simulink model "absbrake"  (R2024a)
settings: Solver=FixedStepAuto  StartTime=0.0  StopTime=20  FixedStep=0.01  MaxStep=.01  RelTol=1e-3  AbsTol=1e-6
PreLoadFcn:
  | % Load initialization data
  | 
  | sldemo_absdata;
values from neighbouring files (symbols this model uses):
  g = 9.8    [final_abs_code.m]
  J = 5    [final_abs_code.m]
  Kf = 1    [final_abs_code.m]
  m = 400    [final_abs_code.m]
  mu_dry = [0.1 0.3 0.6 0.85 0.9 0.9 0.85 0.7 0.3 0.15 0.1]    [final_abs_code.m]
  mu_icy = [0 0.08 0.10 0.095 0.09 0.088 0.085 0.083 0.08 0.079 0.078 0.077 0.076 0.0755 0.075 0.0745 0.074 0.0735 0.073 0.0725 0.072]    [final_abs_code.m]
  mu_wet = [0 0.68 0.70 0.68 0.65 0.63 0.62 0.61 0.60 0.59 0.58 0.57 0.565 0.56 0.555 0.55 0.548 0.546 0.544 0.542 0.54]    [final_abs_code.m]
  Rr = 0.3    [final_abs_code.m]
  slip_dry = [0 0.05 0.1 0.13 0.15 0.17 0.2 0.3 0.5 0.7 1.0]    [final_abs_code.m]
  slip_icy = [0 0.05 0.10 0.15 0.20 0.25 0.30 0.35 0.40 0.45 0.50 0.55 0.60 0.65 0.70 0.75 0.80 0.85 0.90 0.95 1.0]    [final_abs_code.m]
  slip_wet = [0 0.05 0.10 0.15 0.20 0.25 0.30 0.35 0.40 0.45 0.50 0.55 0.60 0.65 0.70 0.75 0.80 0.85 0.90 0.95 1.0]    [final_abs_code.m]
  v0 = 40    [final_abs_code.m]
undefined symbols (not defined in the file or in its folder): DiscIntNeverNeededParam
libraries: fuzblock x1, slpidlib x1
CloseFcn:
  | % Close the plots that are still open
  | h = findobj(0, 'Name', 'ABS Speeds');
  | if ~isempty(h),
  |   close(h);
  | end;
  | 
  | h = findobj(0, 'Name', 'ABS Slip');
  | if ~isempty(h),
  |   close(h);
  | end;
  | 
  | % Clear initial conditions data to avoid cluttering the workspace
  | 
  | clear g v0 Rr Kf m PBmax TB I slip mu ctrl h;
Description:
  | Modeling an Anti-Lock Braking System (ABS)
  | 
  | *Summary*
  | 
  | This example describes a simple model for an Anti-Lock Braking System
  | (ABS). The model simulates the dynamic behavior of a vehicle
  | under hard braking conditions. The model represents a single wheel, which
  | may be replicated a number of times to create a model for a multi-wheel
  | vehicle.
  | 
  | This model uses the signal logging feature in Simulink(R). You log signals to the
  | MATLAB(R) workspace where you can analyze and view them. You can view
  | the code in sldemo_absbrakeplots.m to see how this is done.
  | 
  | In this model, the wheel speed is calculated in a separate component
  | named sldemo_wheelspeed_absbrake.
  | This component is then referenced using a Model block.  Note that both the
  | top model and the referenced model use a variable step solver, so Simulink
  | will track zero-crossings in the referenced model.
settings Model: FPTRunName=Active  ModifiedByFormat=The MathWorks, Inc.  Creator=The MathWorks, Inc.  LastModifiedBy=The MathWorks, Inc.
settings SolverCC: AutoScaleAbsTol=off  AlgebraicLoopSolver=TrustRegion  MaxZcPerStep=1
settings DataIOCC: SaveFormat=Array  SaveOutput=off  SaveTime=off  ReturnWorkspaceOutputs=off  TimeSaveName=time  SignalLoggingName=sldemo_absbrake_output
settings OptimizationCC: DefaultParameterBehavior=Inlined  UseDivisionForNetSlopeComputation=on  InlineInvariantSignals=on  EnhancedBackFolding=on  PassReuseOutputArgsAs=Individual arguments  ExpressionDepthLimit=2147483647  StateBitsets=on  DataBitsets=on  ZeroExternalMemoryAtStartup=off  ZeroInternalMemoryAtStartup=off  EfficientFloat2IntCast=on  LifeSpan=inf  BufferReusableBoundary=off  OptimizeBlockOrder=speed  DifferentSizesBufferReuse=on  EfficientTunableParamExpr=on
settings DebuggingCC: SignalInfNanChecking=warning  SaveWithParameterizedLinksMsg=none  SigSpecEnsureSampleTimeMsg=none  IntegerOverflowMsg=error  ParameterTunabilityLossMsg=error  UnconnectedInputMsg=warning  UnconnectedOutputMsg=warning  UnconnectedLineMsg=warning  UniqueDataStoreMsg=error  BusObjectLabelMismatch=none  AssertControl=DisableAll  AllowSymbolicDim=off  StateNameClashWarn=warning  SubsystemReferenceDiagnosticForUnitTest=warning  SFUnexpectedBacktrackingDiag=warning  SFNoUnconditionalDefaultTransitionDiag=warning  SFUndirectedBroadcastEventsDiag=error  SFExecutionAtInitializationDiag=none  IntegerSaturationMsg=none  ArithmeticOperatorsInVariantConditions=warning
settings HardwareCC: ProdBitPerPointer=32  ProdBitPerSizeT=32  ProdBitPerPtrDiffT=32  ProdLargestAtomicFloat=None  ProdEndianess=Unspecified  ProdWordSize=32  ProdHWDeviceType=32-bit Generic  TargetBitPerPointer=64  TargetBitPerSizeT=64  TargetBitPerPtrDiffT=64  TargetLongLongMode=on  TargetIntDivRoundTo=Zero  TargetEndianess=LittleEndian  TargetWordSize=64  TargetHWDeviceType=MATLAB Host
settings ModelReferenceCC: UpdateModelReferenceTargets=IfOutOfDate  EnableRefExpFcnMdlSchedulingChecks=on  PropagateSignalLabelsOutOfModel=off
settings SFSimCC: SimUseLocalCustomCode=off  CompileTimeRecursionLimit=0  EnableRuntimeRecursion=off  MATLABDynamicMemAlloc=off  CustomCodeUndefinedFunction=UseInterfaceOnly
settings RTWCC: Description=Embedded Coder  SystemTargetFile=ert.tlc  TemplateMakefile=ert_default_tmf  RTWUseLocalCustomCode=off  GPUComputeCapability=3.5  DLArmComputeVersion=19.05
settings CodeAppCC: ForceParamTrailComments=on  IgnoreCustomStorageClasses=off  IgnoreTestpoints=on  OperatorAnnotations=on  SimulinkDataObjDesc=on  SFDataObjDesc=on  MATLABFcnDesc=on  InsertBlockDesc=on
settings ERTTargetCC: UtilityFuncGeneration=Shared location  GenerateSampleERTMain=on  SupportAbsoluteTime=off  ParenthesesLevel=Standards  CastingMode=Standards  GenerateSharedConstants=off  InlinedParameterPlacement=NonHierarchical  ERTCustomFileTemplate=example_file_process.tlc  SuppressUnreachableDefaultCases=off  EnableSignedLeftShifts=off  EnableSignedRightShifts=off
settings ConfigComp: CovMetricSettings=dw  CovSaveCumulativeToWorkspaceVar=on  CovSaveSingleToWorkspaceVar=on  CovExternalEMLEnable=off  CovSFcnEnable=off

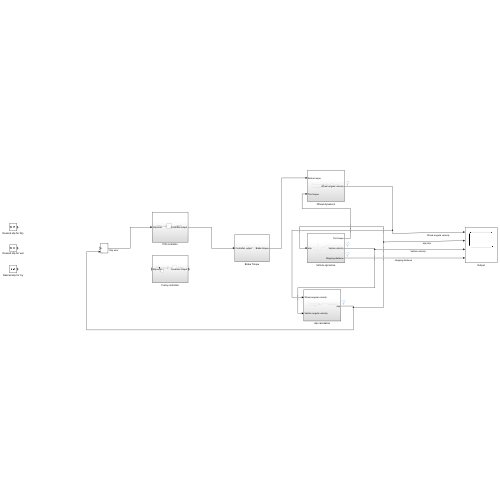
[thumbnail: Simulink's stored preview of the top-level diagram]
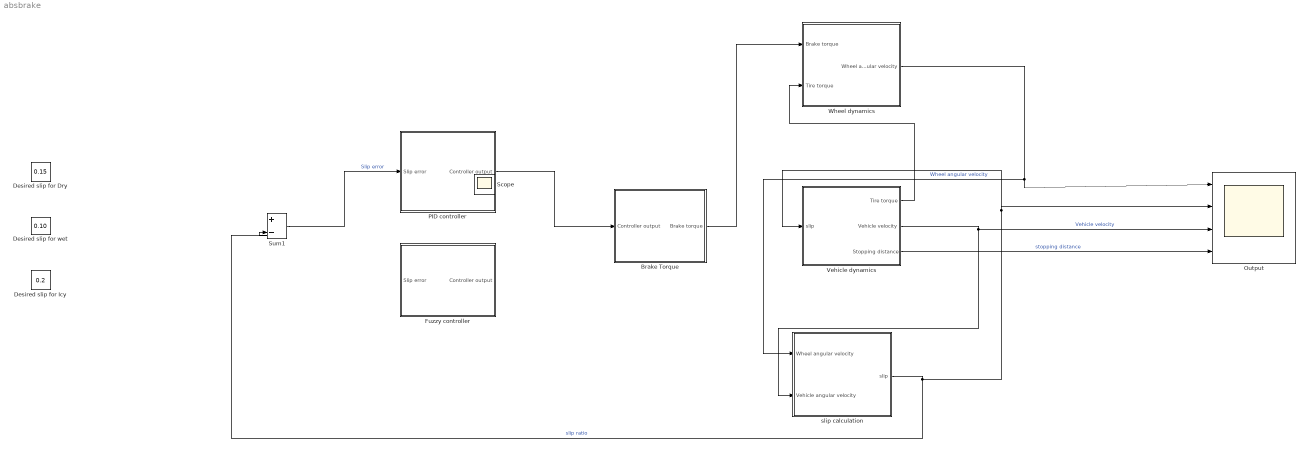
== system absbrake ==
  Brake Torque : Subsystem
  Desired slip for Dry : Constant  Value=0.15
  Desired slip for Icy : Constant  Value=0.2
  Desired slip for wet : Constant  Value=0.10
  Fuzzy controller : Subsystem
  Output : Scope  NumInputPorts=4
  PID controller : Subsystem
  Sum1 : Sum  Inputs=|+-  InputSameDT=on  SaturateOnIntegerOverflow=on  OutDataTypeStr=Inherit: Same as first input
  Vehicle dynamics : Subsystem
  Wheel dynamics : Subsystem
  slip calculation : Subsystem
  Scope : Scope
  wires:
  slip calculation/1(slip) -> Vehicle dynamics/1(slip), Output/2, Sum1/2  "slip ratio"
  Brake Torque/1(Brake torque) -> Wheel dynamics/1(Brake torque)
  Vehicle dynamics/1(Tire torque) -> Wheel dynamics/2(Tire torque)
  Vehicle dynamics/3(Stopping distance) -> Output/4  "stopping distance"
  Vehicle dynamics/2(Vehicle velocity) -> slip calculation/2(Vehicle angular velocity), Output/3  "Vehicle velocity"
  Wheel dynamics/1(Wheel angular velocity) -> Output/1, slip calculation/1(Wheel angular velocity)  "Wheel angular velocity"
  PID controller/1(Controller output) -> Brake Torque/1(Controller output)
  Sum1/1 -> PID controller/1(Slip error)  "Slip error"

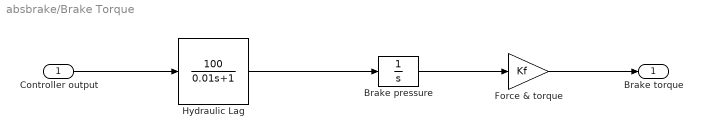
== system absbrake/Brake Torque ==
  Controller output : Inport
  Brake pressure : Integrator  LimitOutput=on  UpperSaturationLimit=1500  LowerSaturationLimit=0
  Force & torque : Gain  Gain=Kf  SaturateOnIntegerOverflow=on  OutDataTypeStr=Inherit: Same as input  ParamDataTypeStr=Inherit: Same as input
  "Hydraulic Lag " : TransferFcn  Numerator=[100]  Denominator=[0.01 1]
  Brake torque : Outport
  wires:
  Controller output/1 -> "Hydraulic Lag "/1
  "Hydraulic Lag "/1 -> Brake pressure/1
  Brake pressure/1 -> Force & torque/1
  Force & torque/1 -> Brake torque/1

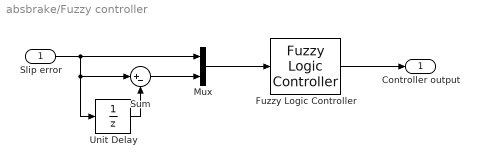
== system absbrake/Fuzzy controller ==
  Slip error : Inport
  Fuzzy Logic Controller : fuzblock/Fuzzy Logic  Controller  FIS='ABS.fis'  OutputSampleNumber=101  DataType=double  FuzzifiedInputs=off  RuleFiringStrengths=off  RuleOutputs=off  AggregatedOutputs=off  SimulateUsing=Interpreted execution  OutOfRangeInputValueMessage=warning  NoRuleFiredMessage=warning  EmptyOutputFuzzySetMessage=warning
  Mux : Mux  Inputs=2
  Sum : Sum  Inputs=|+-
  Unit Delay : UnitDelay  SampleTime=-1  HasFrameUpgradeWarning=on
  Controller output : Outport
  wires:
  Sum/1 -> Mux/2
  Unit Delay/1 -> Sum/2
  Fuzzy Logic Controller/1 -> Controller output/1
  Mux/1 -> Fuzzy Logic Controller/1
  Slip error/1 -> Mux/1, Unit Delay/1, Sum/1

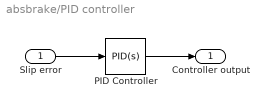
== system absbrake/PID controller ==
  Slip error : Inport
  PID Controller : slpidlib/PID Controller  Controller=PID  Form=Parallel  TimeDomain=Continuous-time  UseExternalTs=off  SampleTime=-1  IntegratorMethod=Forward Euler  FilterMethod=Forward Euler  ControllerParametersSource=internal  P=20  I=18  UseKiTs=off  D=2  UseExternalDerivativeSource=off  N=20  UseFilter=on  TunerSelectOption=Transfer Function Based (PID Tuner App)  InitialConditionSource=internal  InitialConditionForIntegrator=0  InitialConditionForFilter=0  DifferentiatorICPrevScaledInput=0  ExternalReset=none  TrackingMode=off  Kt=1  LimitOutput=off  SatLimitsSource=internal  UpperSaturationLimit=inf  LowerSaturationLimit=-inf  LinearizeAsGain=on  AntiWindupMode=none  Kb=1  LimitIntegrator=off  UpperIntegratorSaturationLimit=inf  LowerIntegratorSaturationLimit=-inf  POutMin=[]  POutMax=[]  IOutMin=[]  IOutMax=[]  DOutMin=[]  DOutMax=[]  NOutMin=[]  NOutMax=[]  SumOutMin=[]  SumOutMax=[]  SaturationOutMin=[]  SaturationOutMax=[]  PParamMin=[]  PParamMax=[]  IParamMin=[]  IParamMax=[]  DParamMin=[]  DParamMax=[]  NParamMin=[]  NParamMax=[]  KbParamMin=[]  KbParamMax=[]  KtParamMin=[]  KtParamMax=[]  KbOutMin=[]  KbOutMax=[]  KtOutMin=[]  KtOutMax=[]  IntegratorOutMin=[]  IntegratorOutMax=[]  FilterOutMin=[]  FilterOutMax=[]  SumI1OutMin=[]  SumI1OutMax=[]  SumI2OutMin=[]  SumI2OutMax=[]  SumI3OutMin=[]  SumI3OutMax=[]  SumI4OutMin=[]  SumI4OutMax=[]  SumDOutMin=[]  SumDOutMax=[]  DifferentiatorOutMin=[]  DifferentiatorOutMax=[]  FilterDiffOutCoefMin=[]  FilterDiffOutCoefMax=[]  ReciprocalOutMin=[]  ReciprocalOutMax=[]  SumDenOutMin=[]  SumDenOutMax=[]  SumNumOutMin=[]  SumNumOutMax=[]  DivideOutMin=[]  DivideOutMax=[]  UdiffTsProdOutMin=[]  UdiffTsProdOutMax=[]  NTsProdOutMin=[]  NTsProdOutMax=[]  UintegralTsProdOutMin=[]  UintegralTsProdOutMax=[]  UngainTsProdOutMin=[]  UngainTsProdOutMax=[]  ClampingZeroOutDataTypeStr=Inherit: Inherit via back propagation  ClampingZeroOutMin=[]  ClampingZeroOutMax=[]  FilterDenConstantOutDataTypeStr=Inherit: Inherit via back propagation  FilterDenConstantOutMin=[]  FilterDenConstantOutMax=[]  PCopyOutDataTypeStr=Inherit: Inherit via back propagation  PCopyOutMin=[]  PCopyOutMax=[]  NCopyOutDataTypeStr=Inherit: Inherit via back propagation  NCopyOutMin=[]  NCopyOutMax=[]  IntegratorContinuousStateAttributes=''  IntegratorStateMustResolveToSignalObject=off  IntegratorRTWStateStorageClass=Auto  FilterContinuousStateAttributes=''  FilterStateMustResolveToSignalObject=off  FilterRTWStateStorageClass=Auto  ParallelPVariant=InternalParameters  IdealPVariant=Disabled  IVariant=InternalParameters  DVariant=InternalParameters  IntegratorVariant=Continuous  SatVariant=Disabled  AWVariant=Passthrough  PCopyVariant=Disabled  TRVariant=Disabled  FdbkBlocksVariant=Forward  IdealPFdbkVariant=Disabled  SatFdbkVariant=Disabled  DerivativeFilterVariant=ContFilter  NVariant=InternalParameters  NCopyVariant=Disabled  FilterICVariant=InternalICsFilter  IntegratorICVariant=InternalICs  ExternalResetVariant=Disabled  TRSumVariant=Passthrough  SumFdbkVariant=Disabled  SumVariant=Sum_PID  TsampFilterVariant=InternalTs  TsampNgainVariant=Passthrough  TsampIntegralVariant=Disabled_SignalSpec  ExternalSaturationOutDataTypeStr=Inherit: Same as second input  DerivativeSourceVariant=ErrorSignal
  Controller output : Outport
  wires:
  Slip error/1 -> PID Controller/1
  PID Controller/1 -> Controller output/1

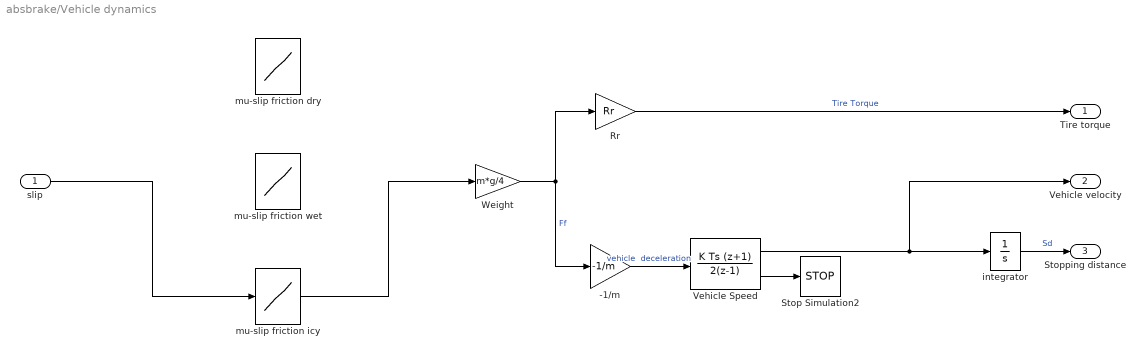
== system absbrake/Vehicle dynamics ==
  slip : Inport
  -1/m : Gain  Gain=-1/m  SaturateOnIntegerOverflow=on  OutDataTypeStr=Inherit: Same as input  ParamDataTypeStr=Inherit: Same as input
  Rr : Gain  Gain=Rr  SaturateOnIntegerOverflow=on  OutDataTypeStr=Inherit: Same as input  ParamDataTypeStr=Inherit: Same as input
  Stop Simulation2 : Stop
  Vehicle Speed : DiscreteIntegrator  IntegratorMethod=Integration: Trapezoidal  InitialCondition=v0  SampleTime=-1  LimitOutput=on  UpperSaturationLimit=1000  LowerSaturationLimit=0  ShowSaturationPort=on  ICPrevOutput=DiscIntNeverNeededParam  ICPrevScaledInput=DiscIntNeverNeededParam
  Weight : Gain  Gain=m*g/4  SaturateOnIntegerOverflow=on  OutDataTypeStr=Inherit: Same as input  ParamDataTypeStr=Inherit: Same as input
  integrator : Integrator  UpperSaturationLimit=1000  LowerSaturationLimit=0
  mu-slip friction dry : Lookup_n-D  NumberOfTableDimensions=1  BreakpointsForDimension1=slip_dry  Table=mu_dry  SaturateOnIntegerOverflow=on
  mu-slip friction icy : Lookup_n-D  NumberOfTableDimensions=1  BreakpointsForDimension1=slip_icy  Table=mu_icy  SaturateOnIntegerOverflow=on
  mu-slip friction wet : Lookup_n-D  NumberOfTableDimensions=1  BreakpointsForDimension1=slip_wet  Table=mu_wet  SaturateOnIntegerOverflow=on
  Tire torque : Outport
  Vehicle velocity : Outport  Port=2
  Stopping distance : Outport  Port=3
  wires:
  Vehicle Speed/1 -> Vehicle velocity/1, integrator/1
  -1/m/1 -> Vehicle Speed/1  "vehicle  deceleration"
  Weight/1 -> Rr/1, -1/m/1  "Ff"
  integrator/1 -> Stopping distance/1  "Sd"
  Vehicle Speed/2 -> Stop Simulation2/1
  Rr/1 -> Tire torque/1  "Tire Torque"
  slip/1 -> mu-slip friction icy/1
  mu-slip friction icy/1 -> Weight/1

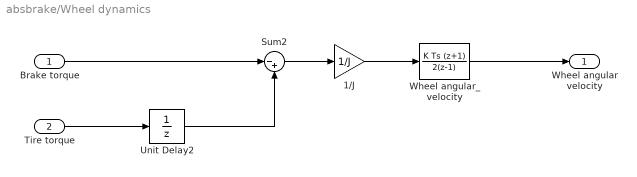
== system absbrake/Wheel dynamics ==
  Brake torque : Inport
  Tire torque : Inport  Port=2
  1/J : Gain  Gain=1/J  SaturateOnIntegerOverflow=on  OutDataTypeStr=Inherit: Same as input  ParamDataTypeStr=Inherit: Same as input
  Sum2 : Sum  Inputs=|-+  InputSameDT=on  SaturateOnIntegerOverflow=on  OutDataTypeStr=Inherit: Same as first input
  Unit Delay2 : UnitDelay  SampleTime=-1  HasFrameUpgradeWarning=on
  Wheel angular_velocity : DiscreteIntegrator  IntegratorMethod=Integration: Trapezoidal  InitialCondition=v0/Rr  SampleTime=-1  LimitOutput=on  UpperSaturationLimit=1000  LowerSaturationLimit=0  ICPrevOutput=DiscIntNeverNeededParam  ICPrevScaledInput=DiscIntNeverNeededParam
  Wheel angular velocity : Outport
  wires:
  Unit Delay2/1 -> Sum2/2
  1/J/1 -> Wheel angular_velocity/1
  Sum2/1 -> 1/J/1
  Wheel angular_velocity/1 -> Wheel angular velocity/1
  Tire torque/1 -> Unit Delay2/1
  Brake torque/1 -> Sum2/1

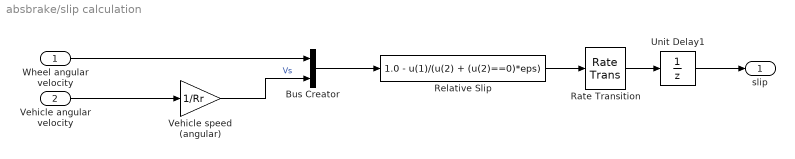
== system absbrake/slip calculation ==
  Wheel angular velocity : Inport
  Vehicle angular velocity : Inport  Port=2
  Bus Creator : BusCreator  Inputs=2
  Rate Transition : RateTransition  OutPortSampleTimeOpt=Inherit
  Relative Slip : Fcn  Expr=1.0 - u(1)/(u(2) + (u(2)==0)*eps)
  Unit Delay1 : UnitDelay  SampleTime=-1  HasFrameUpgradeWarning=on
  Vehicle speed (angular) : Gain  Gain=1/Rr  SaturateOnIntegerOverflow=on  OutDataTypeStr=Inherit: Same as input  ParamDataTypeStr=Inherit: Same as input
  slip : Outport
  wires:
  Unit Delay1/1 -> slip/1
  Rate Transition/1 -> Unit Delay1/1
  Relative Slip/1 -> Rate Transition/1
  Wheel angular velocity/1 -> Bus Creator/1
  Bus Creator/1 -> Relative Slip/1
  Vehicle angular velocity/1 -> Vehicle speed (angular)/1
  Vehicle speed (angular)/1 -> Bus Creator/2  "Vs"
